simulink model "E3"  (R2024a)
settings: Solver=VariableStepAuto  StartTime=0.0  StopTime=10.0  RelTol=1e-3
undefined symbols (not defined in the file): Ad, Bd, Cd, K, kalmf, L, Nd, R_1, R_2
settings Model: Creator=adhish  LastModifiedBy=adhish

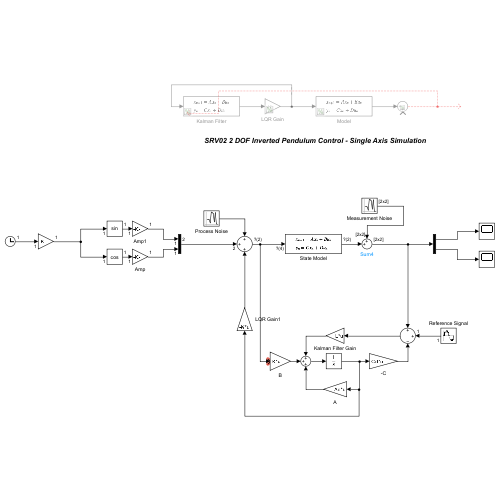
[thumbnail: Simulink's stored preview of the top-level diagram]
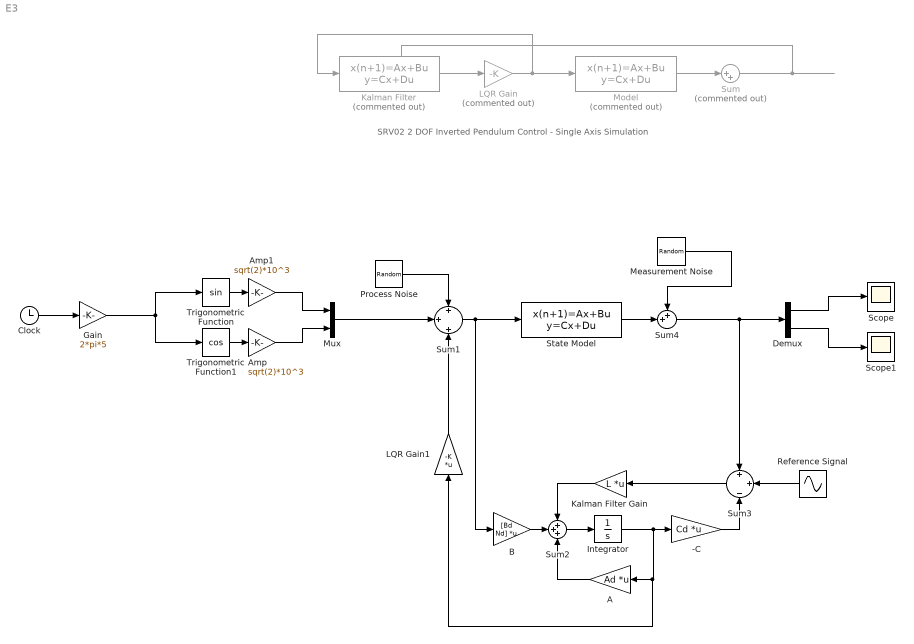
== system E3 ==
  note: SRV02 2 DOF Inverted Pendulum Control - Single Axis Simulation
  -C : Gain  Gain=Cd  Multiplication=Matrix(K*u)
  A : Gain  Gain=Ad  Multiplication=Matrix(K*u)
  Amp : Gain  Gain=sqrt(2)*10^3
  Amp1 : Gain  Gain=sqrt(2)*10^3
  B : Gain  Gain=[Bd Nd]  Multiplication=Matrix(K*u)
  Clock : Clock
  Demux : Demux  Outputs=2
  Gain : Gain  Gain=2*pi*5
  Integrator : Integrator
  Kalman Filter : DiscreteStateSpace  Commented=on  A=kalmf.A  B=kalmf.B  C=kalmf.C  D=kalmf.D  SampleTime=0.005  StateName=Kalman Filter
  Kalman Filter Gain : Gain  Gain=L  Multiplication=Matrix(K*u)
  LQR Gain : Gain  Commented=on  Gain=-K
  LQR Gain1 : Gain  Gain=-K  Multiplication=Matrix(K*u)  SaturateOnIntegerOverflow=on  OutDataTypeStr=Inherit: Same as input  ParamDataTypeStr=Inherit: Same as input
  Measurement Noise : RandomNumber  Variance=R_2  SampleTime=0.005
  Model : DiscreteStateSpace  Commented=on  A=Ad  B=[Bd Nd]  C=Cd  D=zeros(2,4)  SampleTime=0.005
  Mux : Mux  Inputs=2
  Process Noise : RandomNumber  Variance=R_1  SampleTime=0.005
  Reference Signal : Sin  Amplitude=1000  Frequency=2*pi*5  SampleTime=0.005
  Scope : Scope
  Scope1 : Scope
  State Model : DiscreteStateSpace  A=Ad  B=[Bd Nd]  C=Cd  D=zeros(2,4)  SampleTime=0.005
  Sum : Sum  Commented=on  Inputs=|++
  Sum1 : Sum  Inputs=+|+|+
  Sum2 : Sum  Inputs=+++
  Sum3 : Sum  Inputs=+|+|-
  Sum4 : Sum  Inputs=++|
  Trigonometric Function : Trigonometry
  Trigonometric Function1 : Trigonometry  Operator=cos
  wires:
  Kalman Filter/1 -> LQR Gain/1
  LQR Gain/1 -> Kalman Filter/1, Model/1
  Model/1 -> Sum/1
  Sum/1 -> ?
  Kalman Filter Gain/1 -> Sum2/1
  Sum1/1 -> State Model/1, B/1
  -C/1 -> Sum3/3
  B/1 -> Sum2/2
  LQR Gain1/1 -> Sum1/3
  Sum2/1 -> Integrator/1
  A/1 -> Sum2/3
  Sum3/1 -> Kalman Filter Gain/1
  Integrator/1 -> LQR Gain1/1, A/1, -C/1
  Demux/1 -> Scope/1
  Demux/2 -> Scope1/1
  Reference Signal/1 -> Sum3/2
  Mux/1 -> Sum1/2
  Clock/1 -> Gain/1
  Trigonometric Function/1 -> Amp1/1
  Trigonometric Function1/1 -> Amp/1
  Gain/1 -> Trigonometric Function/1, Trigonometric Function1/1
  Amp/1 -> Mux/2
  Amp1/1 -> Mux/1
  Process Noise/1 -> Sum1/1
  State Model/1 -> Sum4/2
  Sum4/1 -> Demux/1, Sum3/1
  Measurement Noise/1 -> Sum4/1
